simulink model "hetSuper_V2026a"  (R2026a)
settings: Solver=FixedStepDiscrete  StopTime=0.2  FixedStep=Ts
values from neighbouring files (symbols this model uses):
  D = 20    [param.m]
  fLO = fc_rx + fIF    (= 2340000)    [param.m]
  fsub = [20e3 60e3 100e3]    [param.m]
  phi = -2*pi*fsub*tau    [calibrate_original.m]    (also in param.m = zeros(1,3))
  Ts = 1/Fs    (= 5e-08)    [param.m]
  Ts2 = 1/Fs2    (= 1e-06)    [param.m]
libraries: dsparch4 x3, dspfdesign x2, dspmlti4 x2, commanapbnd3 x2, dspvision x2
settings Model: Creator=matia  LastModifiedBy=felipe

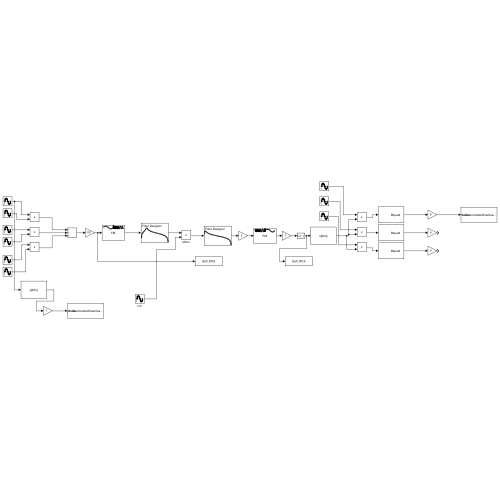
[thumbnail: Simulink's stored preview of the top-level diagram]
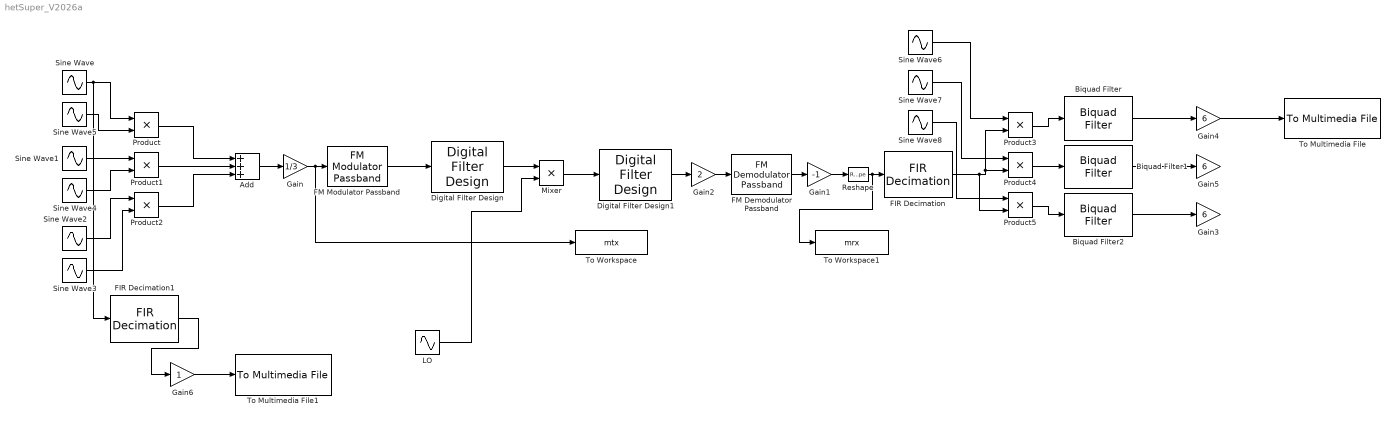
== system hetSuper_V2026a ==
  Add : Sum  Inputs=+++
  Biquad Filter : dsparch4/Biquad Filter  FilterSource=Dialog parameters  CoeffSource=Specify via dialog  FilterObject=BQF  IIRFiltStruct=Direct form II transposed  BiQuadCoeffs=sosAud  ScaleValues=1  IC=0  ICnum=0  ICden=0  a0Flag=Warning  optimizeScaleValues=on  ScaleValueMode=Specify via input port (g)  InputProcessing=Columns as channels (frame based)  roundingMode=Floor  overflowMode=off  scaleValueFracLength=14  denProdOutputFracLength=30  denAccumFracLength=30  secondMemoryFracLength=15
  Biquad Filter1 : dsparch4/Biquad Filter  FilterSource=Dialog parameters  CoeffSource=Specify via dialog  FilterObject=BQF  IIRFiltStruct=Direct form II transposed  BiQuadCoeffs=sosAud  ScaleValues=1  IC=0  ICnum=0  ICden=0  a0Flag=Warning  optimizeScaleValues=on  ScaleValueMode=Specify via input port (g)  InputProcessing=Columns as channels (frame based)  roundingMode=Floor  overflowMode=off  scaleValueFracLength=14  denProdOutputFracLength=30  denAccumFracLength=30  secondMemoryFracLength=15
  Biquad Filter2 : dsparch4/Biquad Filter  FilterSource=Dialog parameters  CoeffSource=Specify via dialog  FilterObject=BQF  IIRFiltStruct=Direct form II transposed  BiQuadCoeffs=sosAud  ScaleValues=1  IC=0  ICnum=0  ICden=0  a0Flag=Warning  optimizeScaleValues=on  ScaleValueMode=Specify via input port (g)  InputProcessing=Columns as channels (frame based)  roundingMode=Floor  overflowMode=off  scaleValueFracLength=14  denProdOutputFracLength=30  denAccumFracLength=30  secondMemoryFracLength=15
  Digital Filter Design : dspfdesign/Digital Filter Design  mwdsp_browser_bugfix_var=off
  Digital Filter Design1 : dspfdesign/Digital Filter Design  mwdsp_browser_bugfix_var=off
  FIR Decimation : dspmlti4/FIR Decimation  FilterSource=Dialog parameters  h=hDec  D=D  filtStruct=Direct form  FilterObject=FDECIM  framing=Enforce single-rate processing  AllowArbitraryInputLength=off  inputOffset=0  outputBufInitCond=0  roundingMode=Floor  overflowMode=off  firstCoeffDataTypeStr=Inherit: Same word length as input  firstCoeffMin=[]  firstCoeffMax=[]  firstCoeffLastDataTypeStr=Inherit: Same word length as input  outputDataTypeStr=Inherit: Same as accumulator  outputMin=[]  outputMax=[]  outputLastDataTypeStr=Inherit: Same as accumulator
  FIR Decimation1 : dspmlti4/FIR Decimation  FilterSource=Dialog parameters  h=hDec  D=D  filtStruct=Direct form  FilterObject=FDECIM  framing=Enforce single-rate processing  AllowArbitraryInputLength=off  inputOffset=0  outputBufInitCond=0  roundingMode=Floor  overflowMode=off  firstCoeffDataTypeStr=Inherit: Same word length as input  firstCoeffMin=[]  firstCoeffMax=[]  firstCoeffLastDataTypeStr=Inherit: Same word length as input  outputDataTypeStr=Inherit: Same as accumulator  outputMin=[]  outputMax=[]  outputLastDataTypeStr=Inherit: Same as accumulator
  FM Demodulator Passband : commanapbnd3/FM Demodulator Passband  Fc=fIF  Ph=0  Kc=df  Ho=1000
  FM Modulator Passband : commanapbnd3/FM Modulator Passband  Fc=fc_rx  Ph=0  Kc=df
  Gain : Gain  Gain=1/3
  Gain1 : Gain  Gain=-1
  Gain2 : Gain  Gain=2
  Gain3 : Gain  Gain=6
  Gain4 : Gain  Gain=6
  Gain5 : Gain  Gain=6
  Gain6 : Gain
  LO : Sin  Frequency=2*pi*fLO  SampleTime=Ts
  Mixer : Product
  Product{,1..5} (6 alike) : Product
  Reshape : Reshape
  Sine Wave : Sin  Frequency=2*pi*2e3  SampleTime=Ts
  Sine Wave1 : Sin  Frequency=2*pi*5e3  SampleTime=Ts
  Sine Wave2 : Sin  Frequency=2*pi*10e3  SampleTime=Ts
  Sine Wave3 : Sin  Frequency=2*pi*100e3  SampleTime=Ts
  Sine Wave4 : Sin  Frequency=2*pi*60e3  SampleTime=Ts
  Sine Wave5 : Sin  Frequency=2*pi*20e3  SampleTime=Ts
  Sine Wave6 : Sin  Frequency=2*pi*fsub(1)  Phase=phi(1)  SampleTime=Ts2
  Sine Wave7 : Sin  Frequency=2*pi*fsub(2)  Phase=phi(2)  SampleTime=Ts2
  Sine Wave8 : Sin  Frequency=2*pi*fsub(3)  Phase=phi(3)  SampleTime=Ts2
  To Multimedia File : dspvision/To Multimedia File  outputFilename=C:\Users\matia\Downloads\3rOutput.wav  streamSelection=Audio only  videoCompressor=None (uncompressed)  audioCompressor=None (uncompressed)  imagePorts=One multidimensional signal  fileType=WAV  audioDatatype=8-bit integer  fourcc=RGB  audioBitRate=128  audioQuality=75  videoQuality=75  mj2000CompFactor=10
      settings: LibrarySourceBlock=audiosinks/To Multimedia File
  To Multimedia File1 : dspvision/To Multimedia File  outputFilename=C:\Users\matia\Downloads\3rOGin.wav  streamSelection=Audio only  videoCompressor=None (uncompressed)  audioCompressor=None (uncompressed)  imagePorts=One multidimensional signal  fileType=WAV  audioDatatype=8-bit integer  fourcc=RGB  audioBitRate=128  audioQuality=75  videoQuality=75  mj2000CompFactor=10
      settings: LibrarySourceBlock=audiosinks/To Multimedia File
  To Workspace : ToWorkspace  VariableName=mtx  SampleTime=Ts
  To Workspace1 : ToWorkspace  VariableName=mrx  SampleTime=Ts
  wires:
  Product/1 -> Add/1
  Product1/1 -> Add/2
  Product2/1 -> Add/3
  Sine Wave/1 -> Product/1, FIR Decimation1/1
  Sine Wave5/1 -> Product/2
  Sine Wave1/1 -> Product1/1
  Sine Wave4/1 -> Product1/2
  Sine Wave2/1 -> Product2/1
  Sine Wave3/1 -> Product2/2
  Add/1 -> Gain/1
  Gain/1 -> To Workspace/1, FM Modulator Passband/1
  LO/1 -> Mixer/2
  FM Modulator Passband/1 -> Digital Filter Design/1
  Digital Filter Design/1 -> Mixer/1
  Mixer/1 -> Digital Filter Design1/1
  Digital Filter Design1/1 -> Gain2/1
  Gain2/1 -> FM Demodulator Passband/1
  FM Demodulator Passband/1 -> Gain1/1
  FIR Decimation/1 -> Product4/2, Product3/2, Product5/2
  Sine Wave6/1 -> Product3/1
  Sine Wave8/1 -> Product5/1
  Sine Wave7/1 -> Product4/1
  Product3/1 -> Biquad Filter/1
  Product4/1 -> Biquad Filter1/1
  Product5/1 -> Biquad Filter2/1
  Biquad Filter/1 -> Gain4/1
  Biquad Filter1/1 -> Gain5/1
  Biquad Filter2/1 -> Gain3/1
  Gain1/1 -> Reshape/1
  Reshape/1 -> To Workspace1/1, FIR Decimation/1
  Gain6/1 -> To Multimedia File1/1
  Gain4/1 -> To Multimedia File/1
  FIR Decimation1/1 -> Gain6/1
